simulink model "servo_transfer_cell"  (R2026a)
settings: Solver=ode4  StopTime=16  FixedStep=0.002
model workspace (MAT data in the model file):
  brakeDamping = 240
  commandData = [0 0.01 0.02 0.03 0.04 0.05 0.06 0.07 0.08 0.09 0.1 0.11 ... (17611 elements, 1601x11)]
  params = [0.01 8 6 1.5 35 0.45 0.8 2 75 110 10 0.65 0.004 0.012 0.12 8 3 240]
  plantCoulomb = 1.5
  plantMass = 8
  plantViscous = 6
(part 1 of 2)
Description:
  | Virtual commissioning of a servo transfer station. SI units. Software demonstration, not a certified safety controller.
settings Model: Creator=alex  LastModifiedBy=alex

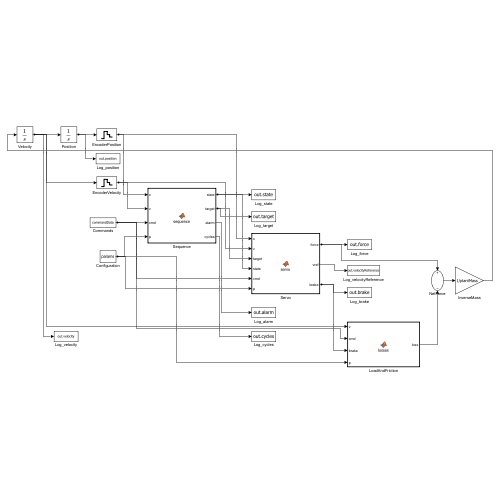
[thumbnail: Simulink's stored preview of the top-level diagram]
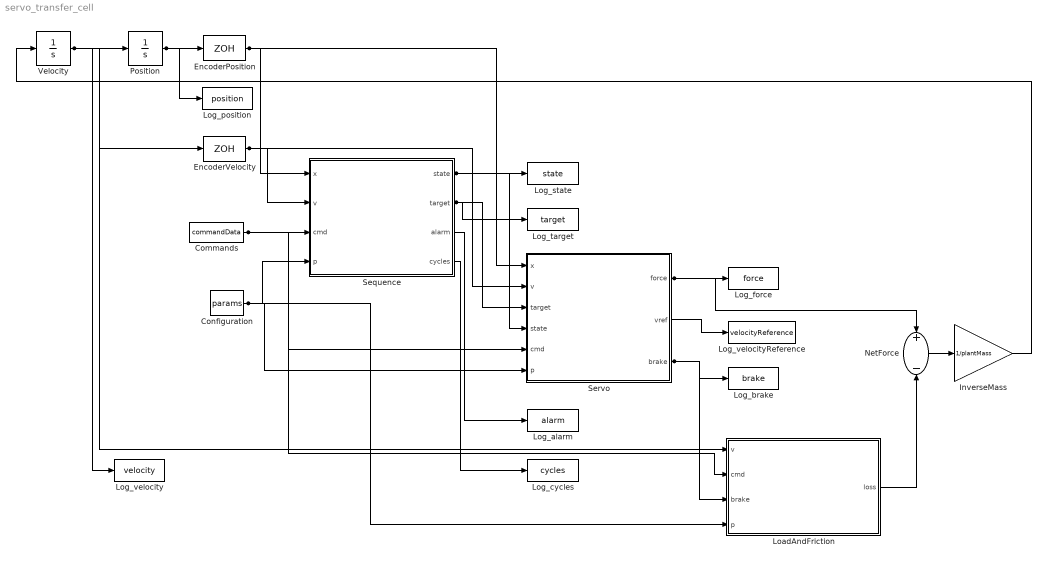
== system servo_transfer_cell ==
  Commands : FromWorkspace  VariableName=commandData  SampleTime=0.01  Interpolate=off  OutputAfterFinalValue=Holding final value
  Configuration : Constant  Value=params
  EncoderPosition : ZeroOrderHold  SampleTime=0.01
  EncoderVelocity : ZeroOrderHold  SampleTime=0.01
  InverseMass : Gain  Gain=1/plantMass
  LoadAndFriction : MATLAB Function  TreatAsAtomicUnit=on
  Log_alarm : ToWorkspace  VariableName=alarm  SaveFormat=Timeseries  SampleTime=-1
  Log_brake : ToWorkspace  VariableName=brake  SaveFormat=Timeseries  SampleTime=-1
  Log_cycles : ToWorkspace  VariableName=cycles  SaveFormat=Timeseries  SampleTime=-1
  Log_force : ToWorkspace  VariableName=force  SaveFormat=Timeseries  SampleTime=-1
  Log_position : ToWorkspace  VariableName=position  SaveFormat=Timeseries  SampleTime=-1
  Log_state : ToWorkspace  VariableName=state  SaveFormat=Timeseries  SampleTime=-1
  Log_target : ToWorkspace  VariableName=target  SaveFormat=Timeseries  SampleTime=-1
  Log_velocity : ToWorkspace  VariableName=velocity  SaveFormat=Timeseries  SampleTime=-1
  Log_velocityReference : ToWorkspace  VariableName=velocityReference  SaveFormat=Timeseries  SampleTime=-1
  NetForce : Sum  Inputs=+-
  Position : Integrator
  Sequence : MATLAB Function  TreatAsAtomicUnit=on
  Servo : MATLAB Function  TreatAsAtomicUnit=on
  Velocity : Integrator
  wires:
  EncoderPosition/1 -> Sequence/1(x), Servo/1(x)
  Velocity/1 -> LoadAndFriction/1(v), Position/1, EncoderVelocity/1, Log_velocity/1
  Sequence/2(target) -> Servo/3(target), Log_target/1
  NetForce/1 -> InverseMass/1
  Position/1 -> EncoderPosition/1, Log_position/1
  EncoderVelocity/1 -> Servo/2(v), Sequence/2(v)
  Commands/1 -> Servo/5(cmd), LoadAndFriction/2(cmd), Sequence/3(cmd)
  Configuration/1 -> Servo/6(p), Sequence/4(p), LoadAndFriction/4(p)
  Sequence/1(state) -> Servo/4(state), Log_state/1
  Sequence/3(alarm) -> Log_alarm/1
  Sequence/4(cycles) -> Log_cycles/1
  Servo/2(vref) -> Log_velocityReference/1
  Servo/1(force) -> NetForce/1, Log_force/1
  Servo/3(brake) -> Log_brake/1, LoadAndFriction/3(brake)
  LoadAndFriction/1(loss) -> NetForce/2
  InverseMass/1 -> Velocity/1
